simulink model "booster_return_3dof"  (R2026a)
settings: Solver=ode45  StopTime=600  MaxStep=0.5  RelTol=1e-9  AbsTol=1e-9
InitFcn:
  | projRoot = fileparts(fileparts(get_param(bdroot,'FileName'))); addpath(genpath(projRoot)); p = vehicleParams(); bb = mission_setup(p);
libraries: aerolibprivatev1p5 x1
settings Model: Creator=Mauro  LastModifiedBy=Mauro

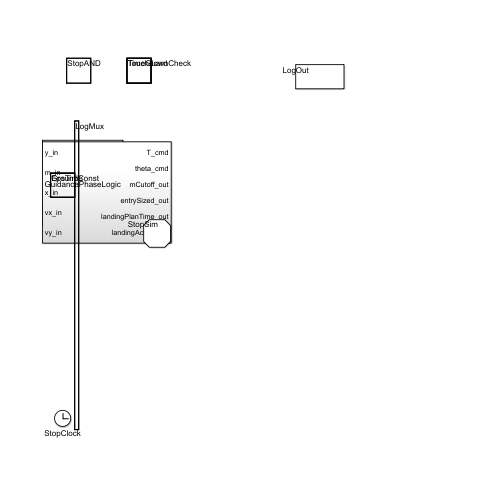
[thumbnail: Simulink's stored preview of the top-level diagram]
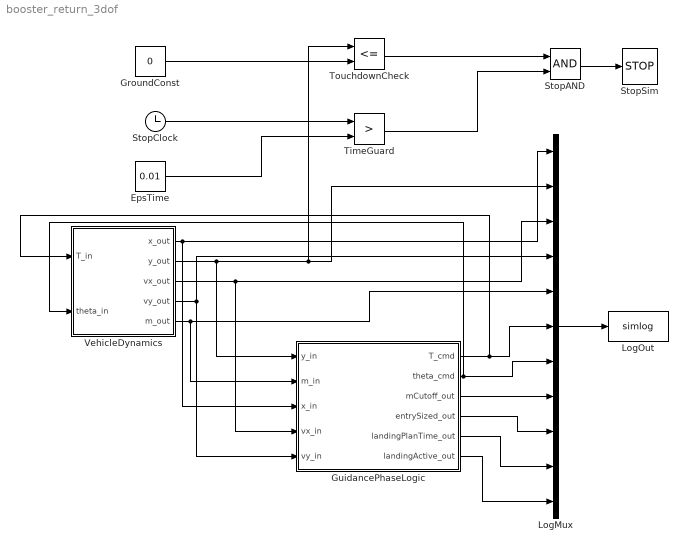
== system booster_return_3dof ==
  EpsTime : Constant  Value=0.01
  GroundConst : Constant  Value=0
  GuidancePhaseLogic : Subsystem
  LogMux : Mux  Inputs=11
  LogOut : ToWorkspace  VariableName=simlog  SaveFormat=Structure With Time  SampleTime=-1
  StopAND : Logic  AllPortsSameDT=off  OutDataTypeStr=boolean
  StopClock : Clock
  StopSim : Stop
  TimeGuard : RelationalOperator  Operator=>  OutDataTypeStr=boolean  RndMeth=Simplest  InputSameDT=off
  TouchdownCheck : RelationalOperator  Operator=<=  OutDataTypeStr=boolean  RndMeth=Simplest  InputSameDT=off
  VehicleDynamics : Subsystem
  wires:
  TimeGuard/1 -> StopAND/2
  VehicleDynamics/2(y_out) -> LogMux/2, TouchdownCheck/1, GuidancePhaseLogic/1(y_in)
  EpsTime/1 -> TimeGuard/2
  StopClock/1 -> TimeGuard/1
  GroundConst/1 -> TouchdownCheck/2
  VehicleDynamics/1(x_out) -> LogMux/1, GuidancePhaseLogic/3(x_in)
  VehicleDynamics/3(vx_out) -> LogMux/3, GuidancePhaseLogic/4(vx_in)
  VehicleDynamics/5(m_out) -> LogMux/5, GuidancePhaseLogic/2(m_in)
  VehicleDynamics/4(vy_out) -> LogMux/4, GuidancePhaseLogic/5(vy_in)
  TouchdownCheck/1 -> StopAND/1
  GuidancePhaseLogic/1(T_cmd) -> VehicleDynamics/1(T_in), LogMux/6
  GuidancePhaseLogic/2(theta_cmd) -> VehicleDynamics/2(theta_in), LogMux/7
  GuidancePhaseLogic/3(mCutoff_out) -> LogMux/8
  GuidancePhaseLogic/4(entrySized_out) -> LogMux/9
  GuidancePhaseLogic/5(landingPlanTime_out) -> LogMux/10
  GuidancePhaseLogic/6(landingActive_out) -> LogMux/11
  StopAND/1 -> StopSim/1
  LogMux/1 -> LogOut/1

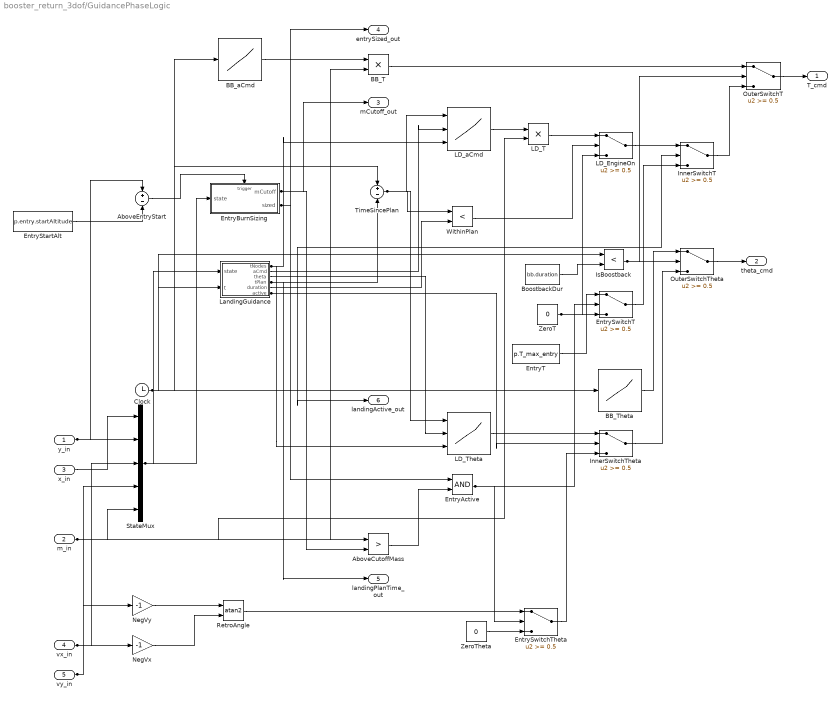
== system booster_return_3dof/GuidancePhaseLogic ==
  y_in : Inport
  m_in : Inport  Port=2
  x_in : Inport  Port=3
  vx_in : Inport  Port=4
  vy_in : Inport  Port=5
  AboveCutoffMass : RelationalOperator  Operator=>  OutDataTypeStr=boolean  RndMeth=Simplest  InputSameDT=off
  AboveEntryStart : Sum  Inputs=+-
  BB_T : Product
  BB_Theta : Lookup_n-D  NumberOfTableDimensions=1  BreakpointsForDimension1=bb.t  Table=bb.theta  InterpMethod=Flat  ExtrapMethod=Clip  InternalRulePriority=Speed  RndMeth=Simplest
  BB_aCmd : Lookup_n-D  NumberOfTableDimensions=1  BreakpointsForDimension1=bb.t  Table=bb.aCmd  InterpMethod=Flat  ExtrapMethod=Clip  InternalRulePriority=Speed  RndMeth=Simplest
  BoostbackDur : Constant  Value=bb.duration
  Clock : Clock
  EntryActive : Logic  AllPortsSameDT=off  OutDataTypeStr=boolean
  EntryBurnSizing : Subsystem  TreatAsAtomicUnit=on
  EntryStartAlt : Constant  Value=p.entry.startAltitude
  EntrySwitchT : Switch  Threshold=0.5  SaturateOnIntegerOverflow=off  InputSameDT=off
  EntrySwitchTheta : Switch  Threshold=0.5  SaturateOnIntegerOverflow=off  InputSameDT=off
  EntryT : Constant  Value=p.T_max_entry
  InnerSwitchT : Switch  Threshold=0.5  SaturateOnIntegerOverflow=off  InputSameDT=off
  InnerSwitchTheta : Switch  Threshold=0.5  SaturateOnIntegerOverflow=off  InputSameDT=off
  IsBoostback : RelationalOperator  Operator=<  OutDataTypeStr=boolean  RndMeth=Simplest  InputSameDT=off
  LD_EngineOn : Switch  Threshold=0.5  SaturateOnIntegerOverflow=off  InputSameDT=off
  LD_T : Product
  LD_Theta : Lookup_n-D  NumberOfTableDimensions=1  BreakpointsForDimension1Source=Input port  BreakpointsForDimension1=[-5:5]  TableSource=Input port  Table=tanh([-5:5])  InterpMethod=Flat  ExtrapMethod=Clip  InternalRulePriority=Speed  RndMeth=Simplest
      settings: InputPortMap=u0,p221,p5
  LD_aCmd : Lookup_n-D  NumberOfTableDimensions=1  BreakpointsForDimension1Source=Input port  BreakpointsForDimension1=[-5:5]  TableSource=Input port  Table=tanh([-5:5])  InterpMethod=Flat  ExtrapMethod=Clip  InternalRulePriority=Speed  RndMeth=Simplest
      settings: InputPortMap=u0,p221,p5
  LandingGuidance : MATLAB Function  TreatAsAtomicUnit=on
  NegVx : Gain  Gain=-1
  NegVy : Gain  Gain=-1
  OuterSwitchT : Switch  Threshold=0.5  SaturateOnIntegerOverflow=off  InputSameDT=off
  OuterSwitchTheta : Switch  Threshold=0.5  SaturateOnIntegerOverflow=off  InputSameDT=off
  RetroAngle : Trigonometry  Operator=atan2
  StateMux : Mux  Inputs=5
  TimeSincePlan : Sum  Inputs=+-
  WithinPlan : RelationalOperator  Operator=<  OutDataTypeStr=boolean  RndMeth=Simplest  InputSameDT=off
  ZeroT : Constant  Value=0
  ZeroTheta : Constant  Value=0
  T_cmd : Outport
  theta_cmd : Outport  Port=2
  mCutoff_out : Outport  Port=3
  entrySized_out : Outport  Port=4
  landingPlanTime_out : Outport  Port=5
  landingActive_out : Outport  Port=6
  wires:
  StateMux/1 -> EntryBurnSizing/1(state), LandingGuidance/1(state)
  AboveEntryStart/1 -> EntryBurnSizing/Trigger
  EntryStartAlt/1 -> AboveEntryStart/2
  vy_in/1 -> StateMux/4, NegVy/1
  vx_in/1 -> StateMux/3, NegVx/1
  LD_Theta/1 -> InnerSwitchTheta/1
  TimeSincePlan/1 -> LD_Theta/1, LD_aCmd/1, WithinPlan/1
  m_in/1 -> BB_T/2, AboveCutoffMass/1, LD_T/2, StateMux/5
  WithinPlan/1 -> LD_EngineOn/2
  x_in/1 -> StateMux/1
  y_in/1 -> AboveEntryStart/1, StateMux/2
  Clock/1 -> IsBoostback/1, BB_aCmd/1, BB_Theta/1, LandingGuidance/2(t), TimeSincePlan/1
  NegVy/1 -> RetroAngle/1
  OuterSwitchTheta/1 -> theta_cmd/1
  BB_T/1 -> OuterSwitchT/1
  NegVx/1 -> RetroAngle/2
  BB_aCmd/1 -> BB_T/1
  EntryBurnSizing/1(mCutoff) -> AboveCutoffMass/2, mCutoff_out/1
  LD_EngineOn/1 -> InnerSwitchT/1
  EntryBurnSizing/2(sized) -> entrySized_out/1, EntryActive/1
  LandingGuidance/1(tNodes) -> LD_Theta/3, LD_aCmd/3
  LandingGuidance/2(aCmd) -> LD_aCmd/2
  LandingGuidance/3(theta) -> LD_Theta/2
  LandingGuidance/4(tPlan) -> TimeSincePlan/2, landingPlanTime_out/1
  LandingGuidance/5(duration) -> WithinPlan/2
  LandingGuidance/6(active) -> InnerSwitchT/2, InnerSwitchTheta/2, landingActive_out/1
  InnerSwitchT/1 -> OuterSwitchT/3
  RetroAngle/1 -> EntrySwitchTheta/1
  EntryActive/1 -> EntrySwitchT/2, EntrySwitchTheta/2
  AboveCutoffMass/1 -> EntryActive/2
  LD_aCmd/1 -> LD_T/1
  ZeroTheta/1 -> EntrySwitchTheta/3
  LD_T/1 -> LD_EngineOn/1
  BoostbackDur/1 -> IsBoostback/2
  EntrySwitchT/1 -> InnerSwitchT/3
  ZeroT/1 -> EntrySwitchT/3, LD_EngineOn/3
  EntryT/1 -> EntrySwitchT/1
  EntrySwitchTheta/1 -> InnerSwitchTheta/3
  BB_Theta/1 -> OuterSwitchTheta/1
  IsBoostback/1 -> OuterSwitchT/2, OuterSwitchTheta/2
  InnerSwitchTheta/1 -> OuterSwitchTheta/3
  OuterSwitchT/1 -> T_cmd/1

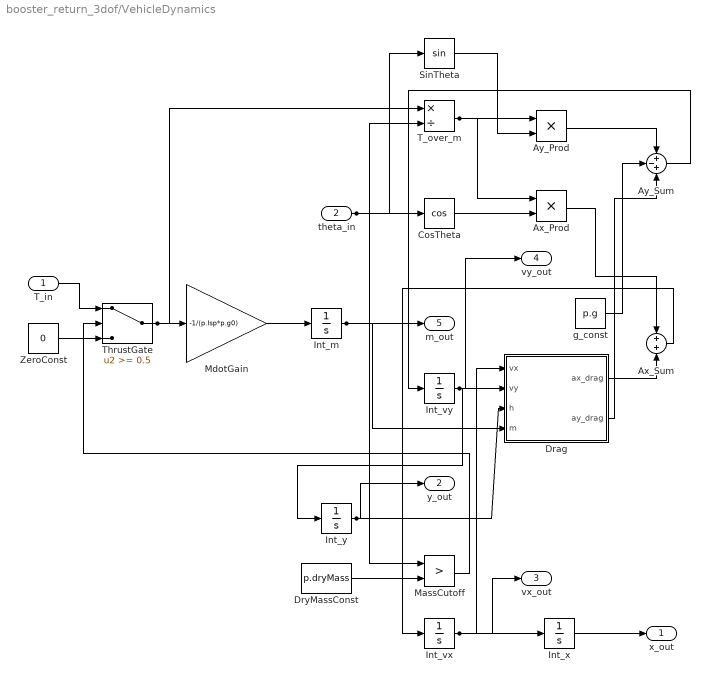
== system booster_return_3dof/VehicleDynamics ==
  T_in : Inport
  theta_in : Inport  Port=2
  Ax_Prod : Product
  Ax_Sum : Sum
  Ay_Prod : Product
  Ay_Sum : Sum  Inputs=+-+
  CosTheta : Trigonometry  Operator=cos
  Drag : Subsystem
  DryMassConst : Constant  Value=p.dryMass
  Int_m : Integrator  InitialCondition=p.m0
  Int_vx : Integrator  InitialCondition=p.sep.vx
  Int_vy : Integrator  InitialCondition=p.sep.vy
  Int_x : Integrator  InitialCondition=p.sep.x
  Int_y : Integrator  InitialCondition=p.sep.y
  MassCutoff : RelationalOperator  Operator=>  OutDataTypeStr=boolean  RndMeth=Simplest  InputSameDT=off
  MdotGain : Gain  Gain=-1/(p.Isp*p.g0)
  SinTheta : Trigonometry
  T_over_m : Product  Inputs=*/
  ThrustGate : Switch  Threshold=0.5  SaturateOnIntegerOverflow=off  InputSameDT=off
  ZeroConst : Constant  Value=0
  g_const : Constant  Value=p.g
  x_out : Outport
  y_out : Outport  Port=2
  vx_out : Outport  Port=3
  vy_out : Outport  Port=4
  m_out : Outport  Port=5
  wires:
  MassCutoff/1 -> ThrustGate/2
  T_in/1 -> ThrustGate/1
  DryMassConst/1 -> MassCutoff/2
  ThrustGate/1 -> T_over_m/1, MdotGain/1
  ZeroConst/1 -> ThrustGate/3
  MdotGain/1 -> Int_m/1
  theta_in/1 -> CosTheta/1, SinTheta/1
  Int_y/1 -> Drag/3(h), y_out/1
  Int_m/1 -> Drag/4(m), MassCutoff/1, m_out/1, T_over_m/2
  Ax_Prod/1 -> Ax_Sum/1
  Ay_Prod/1 -> Ay_Sum/1
  SinTheta/1 -> Ay_Prod/2
  T_over_m/1 -> Ax_Prod/1, Ay_Prod/1
  CosTheta/1 -> Ax_Prod/2
  Drag/2(ay_drag) -> Ay_Sum/3
  Int_vy/1 -> Int_y/1, vy_out/1, Drag/2(vy)
  Int_vx/1 -> Int_x/1, vx_out/1, Drag/1(vx)
  Ax_Sum/1 -> Int_vx/1
  Ay_Sum/1 -> Int_vy/1
  g_const/1 -> Ay_Sum/2
  Drag/1(ax_drag) -> Ax_Sum/2
  Int_x/1 -> x_out/1

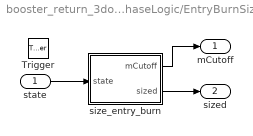
== system booster_return_3dof/GuidancePhaseLogic/EntryBurnSizing ==
  state : Inport
  Trigger : TriggerPort  TriggerType=falling  VariantControl=(inherit)
  size_entry_burn : MATLAB Function  TreatAsAtomicUnit=on
  mCutoff : Outport
  sized : Outport  Port=2
  wires:
  state/1 -> size_entry_burn/1(state)
  size_entry_burn/2(sized) -> sized/1
  size_entry_burn/1(mCutoff) -> mCutoff/1

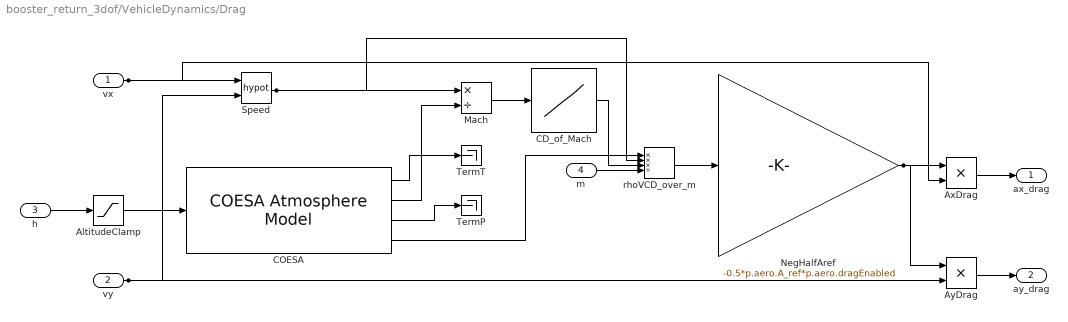
== system booster_return_3dof/VehicleDynamics/Drag ==
  vx : Inport
  vy : Inport  Port=2
  h : Inport  Port=3
  m : Inport  Port=4
  AltitudeClamp : Saturate  UpperLimit=p.atmo.maxAltitude  LowerLimit=0
  AxDrag : Product
  AyDrag : Product
  CD_of_Mach : Lookup_n-D  NumberOfTableDimensions=1  BreakpointsForDimension1=p.aero.mach  Table=p.aero.CD  ExtrapMethod=Clip  InternalRulePriority=Speed  RndMeth=Simplest
  COESA : aerolibprivatev1p5/COESA Atmosphere Model  units=Metric
  Mach : Product  Inputs=*/
  NegHalfAref : Gain  Gain=-0.5*p.aero.A_ref*p.aero.dragEnabled
  Speed : Math  Operator=hypot
  TermP : Terminator
  TermT : Terminator
  rhoVCD_over_m : Product  Inputs=***/
  ax_drag : Outport
  ay_drag : Outport  Port=2
  wires:
  Speed/1 -> rhoVCD_over_m/2, Mach/1
  AltitudeClamp/1 -> COESA/1
  vx/1 -> AxDrag/2, Speed/1
  h/1 -> AltitudeClamp/1
  vy/1 -> Speed/2, AyDrag/2
  COESA/3 -> TermP/1
  COESA/2 -> Mach/2
  COESA/1 -> TermT/1
  COESA/4 -> rhoVCD_over_m/1
  NegHalfAref/1 -> AxDrag/1, AyDrag/1
  Mach/1 -> CD_of_Mach/1
  CD_of_Mach/1 -> rhoVCD_over_m/3
  m/1 -> rhoVCD_over_m/4
  rhoVCD_over_m/1 -> NegHalfAref/1
  AxDrag/1 -> ax_drag/1
  AyDrag/1 -> ay_drag/1

== matlab function booster_return_3dof/GuidancePhaseLogic/LandingGuidance ==
  settings: updateMethod=DISCRETE  sampleTime=p.landing.loopPeriod
  data: state input; tNodes output size=[p.landing.N-1 1]; t input; aCmd output size=[p.landing.N-1 1]; theta output size=[p.landing.N-1 1]; tPlan output size=1; duration output size=1; active output size=1; p parameter
function [tNodes, aCmd, theta, tPlan, duration, active] = landing_guidance(state, t, p)
%LANDING_GUIDANCE In-flight landing guidance: plan at ignition, then
%   re-plan periodically (warm-started) until the final window. Keeps the
%   current plan as persistent arrays; the guidance itself runs as MATLAB
%   code (extrinsic), so this block is simulation-only.
coder.extrinsic('landing_replan');
N = p.landing.N; K = N - 1;
persistent planned pX pU pS pM0 pT pA pTh pDur pTPlan pTLast
if isempty(planned)
    planned = false; pX = zeros(5, N); pU = zeros(3, K); pS = 0; pM0 = 0;
    pT = (0:K-1)'; pA = zeros(K, 1); pTh = zeros(K, 1);
    pDur = 0; pTPlan = 0; pTLast = -1e9;
end
doSolve = false; warm = false;
if ~planned
    doSolve = state(2) <= p.landingIgniteAltitude && state(4) < 0;
else
    remaining = pDur - (t - pTPlan);
    if remaining > p.landing.freezeTime && state(2) > p.landing.minReplanAltitude ...
            && (t - pTLast) >= p.landing.replanPeriod - 1e-9
        doSolve = true; warm = true;
    end
end
if doSolve
    Xs = zeros(5, N); Us = zeros(3, K); s = 0; m0 = 0;
    tn = zeros(K, 1); a = zeros(K, 1); th = zeros(K, 1); dur = 0; ok = false;
    [Xs, Us, s, m0, tn, a, th, dur, ok] = landing_replan(state, p, warm, pX, pU, pS, pM0, t - pTPlan);
    pTLast = t;
    if ok
        planned = true; pX = Xs; pU = Us; pS = s; pM0 = m0;
        pT = tn; pA = a; pTh = th; pDur = dur; pTPlan = t;
    end
end
tNodes = pT; aCmd = pA; theta = pTh; tPlan = pTPlan; duration = pDur;
active = double(planned);

== matlab function booster_return_3dof/GuidancePhaseLogic/EntryBurnSizing/size_entry_burn ==
  data: state input; mCutoff output; sized output; p parameter
function [mCutoff, sized] = size_entry_burn(state, p)
%SIZE_ENTRY_BURN Runs once, when the stage descends through the entry
%   start altitude: sizes the entry burn from the measured state with
%   the guidance's own predictor (entry_burn_sizing, MATLAB code run
%   extrinsically) and returns the engine-cutoff mass.
coder.extrinsic('entry_cutoff_mass');
mCutoff = 0;
sized = 0;
if p.entry.enabled
    mCutoff = entry_cutoff_mass(state, p);
    sized = 1;
end
